simulink model "rfsoc4x2_ospfb_128"  (R2021a)
(part 3 of 339)

  pipeline45/1(q) -> q14/3(we)
  pipeline50/1(q) -> q15/1(addr)
  pipeline9/1(q) -> simple_bram_vacc3/1(new_acc)
  pipeline37/1(q) -> simple_bram_vacc1/2(din)
  Reinterpret5/1 -> pipeline11/1(d)
  Delay55/1 -> Delay92/1
  Reinterpret4/1 -> pipeline7/1(d)
  pipeline40/1(q) -> simple_bram_vacc5/1(new_acc)
  pipeline23/1(q) -> pipeline15/1(d)
  power8/1 -> Delay40/1
  Delay41/1 -> pipeline12/1(d)
  fft2/4(out02) -> Delay38/1
  pipeline43/1(q) -> simple_bram_vacc6/2(din)
  simple_bram_vacc6/2(valid) -> pipeline45/1(d)
  pipeline7/1(q) -> q16/2(data_in)
  Delay97/1 -> pipeline70/1(d)
  Delay91/1 -> pipeline39/1(d)
  q9/1(data_out) -> Terminator17/1
  Delay46/1 -> power8/1
  simple_bram_vacc4/2(valid) -> pipeline52/1(d)
  Delay93/1 -> pipeline8/1(d)
  [new_acc] -> pipeline9/1(d)
  simple_bram_vacc7/1(dout) -> Reinterpret2/1
  fft2/3(out01) -> Delay36/1
  fft2/7(out05) -> Delay53/1
  simple_bram_vacc6/1(dout) -> Reinterpret6/1
  pipeline51/1(q) -> q15/2(data_in)
  pipeline47/1(q) -> pipeline41/1(d)
  [new_acc] -> pipeline32/1(d)
  q10/1(data_out) -> Terminator9/1
  Reinterpret8/1 -> pipeline51/1(d)
  pipeline33/1(q) -> simple_bram_vacc2/2(din)
  simple_bram_vacc4/1(dout) -> Reinterpret4/1
  Delay44/1 -> Delay39/1
  q11/1(data_out) -> Terminator10/1
  spect_cnt1/1 -> pipeline29/1(d), pipeline22/1(d), pipeline30/1(d), pipeline53/1(d), pipeline46/1(d), pipeline59/1(d), pipeline50/1(d), pipeline26/1(d)
  Reinterpret2/1 -> pipeline38/1(d)
  [new_acc] -> pipeline16/1(d)
  power6/1 -> Delay97/1
  [new_acc] -> pipeline40/1(d)
  Delay42/1 -> power2/1
  simple_bram_vacc1/2(valid) -> pipeline25/1(d)
  simple_bram_vacc3/1(dout) -> Reinterpret8/1
  Delay92/1 -> power5/1
  Delay32/1 -> Delay44/1
  pipeline6/1(q) -> simple_bram_vacc4/2(din)
  [new_acc] -> pipeline14/1(d)
  [acc_len] -> acc_cntrl1/1(acc_len)
  pipeline5/1(q) -> simple_bram_vacc4/1(new_acc)
  pipeline26/1(q) -> q11/1(addr)
  Delay38/1 -> Delay42/1
  pipeline28/1(q) -> q12/3(we)
  Delay96/1 -> power6/1
  Delay53/1 -> Delay54/1
  fft2/9(out07) -> Delay95/1
  pipeline16/1(q) -> simple_bram_vacc16/1(new_acc)
  Delay48/1 -> power3/1
  pipeline31/1(q) -> pipeline33/1(d)
  Delay40/1 -> pipeline23/1(d)
  Delay52/1 -> Delay94/1
  pipeline25/1(q) -> q11/3(we)
  pipeline32/1(q) -> simple_bram_vacc2/1(new_acc)
  power1/1 -> Delay41/1
  simple_bram_vacc2/1(dout) -> Reinterpret1/1
  Delay35/1 -> Delay46/1
  pipeline8/1(q) -> pipeline10/1(d)
  Delay51/1 -> pipeline31/1(d)
  pipeline15/1(q) -> simple_bram_vacc7/2(din)
  pipeline48/1(q) -> q14/2(data_in)
  power4/1 -> Delay91/1
  power7/1 -> Delay56/1
  simple_bram_vacc5/2(valid) -> pipeline44/1(d)
  simple_bram_vacc5/1(dout) -> Reinterpret5/1
  q13/1(data_out) -> Terminator44/1
  simple_bram_vacc16/1(dout) -> Reinterpret3/1
  power2/1 -> Delay45/1
  fft2/8(out06) -> Delay55/1
  pipeline53/1(q) -> q13/1(addr)
  pipeline42/1(q) -> simple_bram_vacc6/1(new_acc)
  pipeline41/1(q) -> simple_bram_vacc5/2(din)
  q15/1(data_out) -> Terminator36/1
  Delay47/1 -> Delay48/1
  pipeline21/1(q) -> q10/3(we)
  power5/1 -> Delay93/1
  pipeline29/1(q) -> q9/1(addr)
  pipeline39/1(q) -> pipeline43/1(d)
  q14/1(data_out) -> Terminator35/1
  pipeline44/1(q) -> q13/3(we)
  power3/1 -> Delay51/1
  acc_cntrl1/1(new_acc) -> [new_acc]
  Delay95/1 -> Delay96/1
  q12/1(data_out) -> Terminator13/1
  fft2/2(out00) -> Delay35/1
  pipeline36/1(q) -> simple_bram_vacc1/1(new_acc)
  pipeline27/1(q) -> q11/2(data_in)
  Delay37/1 -> power1/1
  munge3/1(dout) -> bus_expand6/1(bus_in)
  bus_expand6/3(out6) -> fft2/5(in02)
  bus_expand6/4(out5) -> fft2/6(in03)
  bus_expand6/6(out3) -> fft2/8(in05)
  bus_expand6/1(msb_out8) -> fft2/3(in00)
  bus_expand6/8(lsb_out1) -> fft2/10(in07)
  [pfb1_sync] -> Delay43/1
  Delay43/1 -> fft2/1(sync)
  Constant60/1 -> fft2/2(shift)
  bus_expand6/7(out2) -> fft2/9(in06)
  fft2/10(of) -> Terminator45/1
  bus_expand6/2(out7) -> fft2/4(in01)
  bus_expand6/5(out4) -> fft2/7(in04)
  Delay31/1 -> Mux4/1
  [ram3_out1] -> Mux4/2
  Mux4/1 -> munge3/1(din)
  [ram3_out8] -> Mux4/9
  [ram3_out2] -> Mux4/3
  [ram3_out4] -> Mux4/5
  [ram3_out7] -> Mux4/8
  [ram3_out5] -> Mux4/6
  [mux_sel] -> Delay31/1
  [ram3_out3] -> Mux4/4
  [ram3_out6] -> Mux4/7
  Constant54/1 -> Dual Port RAM15/6
  Dual Port RAM15/2 -> [ram3_out5]
  Dual Port RAM18/2 -> [ram3_out3]
  [read_addr3] -> Dual Port RAM10/4
  [pfb_out3] -> Dual Port RAM18/2
  [write_addr3] -> Dual Port RAM17/1
  Constant53/1 -> Dual Port RAM15/5
  Constant34/1 -> Dual Port RAM9/6
  Dual Port RAM8/1 -> Terminator15/1
  Dual Port RAM16/1 -> Terminator14/1
  [write_addr3] -> Dual Port RAM18/1
  Constant58/1 -> Dual Port RAM7/5
  Dual Port RAM9/2 -> [ram3_out8]
  [write_addr3] -> Dual Port RAM8/1
  [pfb_out2] -> Dual Port RAM17/2
  Dual Port RAM7/1 -> Terminator5/1
  [read_addr3] -> Dual Port RAM7/4
  Constant33/1 -> Dual Port RAM9/5
  [pfb_out1] -> Dual Port RAM7/2
  Constant52/1 -> Dual Port RAM15/3
  [read_addr3] -> Dual Port RAM9/4
  Constant31/1 -> Dual Port RAM8/6
  Constant57/1 -> Dual Port RAM7/3
  Constant61/1 -> Dual Port RAM17/3
  Constant27/1 -> Dual Port RAM10/6
  [write_addr3] -> Dual Port RAM10/1
  Dual Port RAM8/2 -> [ram3_out7]
  Constant7/1 -> Dual Port RAM8/3
  [pfb_out7] -> Dual Port RAM8/2
  [write_addr3] -> Dual Port RAM16/1
  Dual Port RAM7/2 -> [ram3_out1]
  Dual Port RAM10/1 -> Terminator42/1
  Constant26/1 -> Dual Port RAM10/5
  [pfb_out5] -> Dual Port RAM15/2
  [write_addr3] -> Dual Port RAM9/1
  Constant36/1 -> Dual Port RAM16/6
  Constant22/1 -> Dual Port RAM8/5
  Constant56/1 -> Dual Port RAM17/6
  [read_addr3] -> Dual Port RAM16/4
  Dual Port RAM10/2 -> [ram3_out4]
  Constant23/1 -> Dual Port RAM18/5
  [pfb_out8] -> Dual Port RAM9/2
  Dual Port RAM16/2 -> [ram3_out6]
  Constant32/1 -> Dual Port RAM9/3
  Constant62/1 -> Dual Port RAM16/3
  Dual Port RAM17/2 -> [ram3_out2]
  Dual Port RAM9/1 -> Terminator39/1
  [write_addr3] -> Dual Port RAM7/1
  [read_addr3] -> Dual Port RAM15/4
  Dual Port RAM18/1 -> Terminator41/1
  [read_addr3] -> Dual Port RAM18/4
  Constant59/1 -> Dual Port RAM7/6
  [read_addr3] -> Dual Port RAM17/4
  [write_addr3] -> Dual Port RAM15/1
  Constant5/1 -> Dual Port RAM18/3
  Constant35/1 -> Dual Port RAM16/5
  Constant25/1 -> Dual Port RAM10/3
  [read_addr3] -> Dual Port RAM8/4
  Constant55/1 -> Dual Port RAM17/5
  Dual Port RAM15/1 -> Terminator43/1
  Dual Port RAM17/1 -> Terminator40/1
  [pfb_out6] -> Dual Port RAM16/2
  Constant24/1 -> Dual Port RAM18/6
  [pfb_out4] -> Dual Port RAM10/2
  [pfb1_sync] -> Counter21/1, Counter30/1
  [pfb1_sync] -> Counter22/1
  edge_detect10/1(out) -> Logical1/2
  edge_detect8/1(out) -> Logical6/2
  Counter22/1 -> Delay30/1
  Counter30/1 -> [mux_sel]
  [pfb1_sync] -> Counter28/1, Counter27/1
  Logical5/1 -> Counter26/2
  Counter29/1 -> Slice7/1
  Slice10/1 -> edge_detect10/1(in)
  edge_detect9/1(out) -> Logical7/2
  AddSub4/1 -> [write_addr3]
  [pfb1_sync] -> Counter24/1, Counter23/1
  Counter20/1 -> Delay29/1
  [en_ctrl2] -> Logical7/1
  Counter24/1 -> Slice9/1
  Logical1/1 -> Counter30/2
  [pfb1_sync] -> Counter29/1, Counter26/1
  Counter27/1 -> AddSub4/1
  Slice7/1 -> edge_detect7/1(in)
  [en_ctrl2] -> Logical6/1
  Logical6/1 -> Counter27/2
  [en_ctrl2] -> Logical1/1
  Slice8/1 -> edge_detect8/1(in)
  Counter21/1 -> Slice10/1
  Counter28/1 -> Slice8/1
  [en_ctrl2] -> Logical5/1
  Delay29/1 -> AddSub5/2
  Delay30/1 -> AddSub6/2
  Slice9/1 -> edge_detect9/1(in)
  edge_detect7/1(out) -> Logical5/2
  [pfb1_sync] -> Counter20/1
  Counter26/1 -> AddSub5/1
  AddSub5/1 -> AddSub4/2
  Logical7/1 -> Counter23/2
  AddSub6/1 -> [read_addr3]
  Counter23/1 -> AddSub6/1
  fft_wideband_real1/9(out07) -> Delay28/1
  fft_wideband_real1/8(out06) -> Delay27/1
  Delay24/1 -> [pfb_out5]
  bus_expand5/14(out3) -> fft_wideband_real1/16(in013)
  bus_expand5/10(out7) -> fft_wideband_real1/12(in09)
  bus_expand5/2(out15) -> fft_wideband_real1/4(in01)
  bus_expand5/16(lsb_out1) -> fft_wideband_real1/18(in015)
  Delay19/1 -> [pfb_out2]
  bus_expand5/5(out12) -> fft_wideband_real1/7(in04)
  Delay26/1 -> [pfb_out6]
  [pff1_sync] -> Delay18/1
  Delay27/1 -> [pfb_out7]
  Delay28/1 -> [pfb_out8]
  bus_expand5/11(out6) -> fft_wideband_real1/13(in010)
  Delay20/1 -> [pfb_out3]
  fft_wideband_real1/2(out00) -> Delay7/1
  Delay22/1 -> [pfb_out4]
  bus_expand5/15(out2) -> fft_wideband_real1/17(in014)
  fft_wideband_real1/6(out04) -> Delay24/1
  bus_expand5/4(out13) -> fft_wideband_real1/6(in03)
  fft_wideband_real1/5(out03) -> Delay22/1
  bus_expand5/1(msb_out16) -> fft_wideband_real1/3(in00)
  bus_expand5/6(out11) -> fft_wideband_real1/8(in05)
  bus_expand5/3(out14) -> fft_wideband_real1/5(in02)
  fft_wideband_real1/4(out02) -> Delay20/1
  bus_expand5/12(out5) -> fft_wideband_real1/14(in011)
  Delay18/1 -> fft_wideband_real1/1(sync)
  bus_expand5/7(out10) -> fft_wideband_real1/9(in06)
  [ram2_out] -> bus_expand5/1(bus_in)
  Constant4/1 -> fft_wideband_real1/2(shift)
  fft_wideband_real1/10(of) -> Terminator46/1
  bus_expand5/8(out9) -> fft_wideband_real1/10(in07)
  bus_expand5/9(out8) -> fft_wideband_real1/11(in08)
  fft_wideband_real1/3(out01) -> Delay19/1
  Delay7/1 -> [pfb_out1]
  fft_wideband_real1/1(sync_out) -> [pfb1_sync]
  bus_expand5/13(out4) -> fft_wideband_real1/15(in012)
  fft_wideband_real1/7(out05) -> Delay26/1
  bus_create5/1(bus_out) -> [current_data]
  bus_expand1/1(msb_out12) -> bus_create5/1(in1)
  bus_expand1/2(out11) -> bus_create5/2(in2)
  bus_expand1/3(out10) -> bus_create5/3(in3)
  bus_expand1/4(out9) -> bus_create5/4(in4)
  bus_expand1/5(out8) -> bus_create5/5(in5)
  bus_expand1/6(out7) -> bus_create5/6(in6)
  bus_expand1/7(out6) -> bus_create5/7(in7)
  bus_expand1/8(out5) -> bus_create5/8(in8)
  bus_expand1/9(out4) -> bus_create5/9(in9)
  bus_expand1/10(out3) -> bus_create5/10(in10)
  bus_expand1/11(out2) -> bus_create5/11(in11)
  bus_expand1/12(lsb_out1) -> bus_create5/12(in12)
  Delay102/1 -> AddSub7/1
  munge5/1(dout) -> mux_2/1(bus_in)
  [sync_gen] -> Counter33/1
  Slice13/1 -> Concat3/1
  Delay103/1 -> Relational3/1
  Constant67/1 -> Dual Port RAM19/7
  Dual Port RAM19/1 -> [ram_outa]
  Concat3/1 -> [c2]
  Concat9/1 -> [c3]
  [write_en] -> Logical8/2
  [current_data] -> Delay98/1
  Slice12/1 -> Delay100/1
  Delay98/1 -> Concat2/2
  Counter36/1 -> Slice18/1
  [c1] -> Mux6/3
  [sync_gen] -> Counter34/1
  Counter31/1 -> Delay103/1
  Mux6/1 -> [os_data]
  Constant64/1 -> Relational1/2
  [sync_gen] -> Counter31/1
  Dual Port RAM19/2 -> [ram_outb]
  Constant69/1 -> AddSub8/2
  Convert4/1 -> [en_ctrl]
  [current_data] -> Concat9/1
  Counter35/1 -> AddSub7/2
  Relational2/1 -> Mux7/1
  Constant66/1 -> Dual Port RAM19/6
  [sync_gen] -> Counter32/1
  Counter32/1 -> Delay101/1
  Logical8/1 -> Counter33/2
  Slice11/1 -> Concat2/1
  [os_data] -> Dual Port RAM19/2
  AddSub7/1 -> AddSub8/1, Mux7/2, Relational2/1
  [en_ctrl] -> Logical8/1
  Concat2/1 -> [c1]
  Logical11/1 -> Counter35/2
  Slice14/1 -> Delay99/1
  [write_addr] -> Dual Port RAM19/1
  [current_data] -> Slice14/1, Slice13/1
  Constant68/1 -> Relational2/2
  [read_addr] -> Dual Port RAM19/4
  Relational3/1 -> [ram_out_sel]
  Counter33/1 -> [write_addr]
  Constant65/1 -> Dual Port RAM19/5
  Delay99/1 -> Concat9/2
  [write_en] -> Dual Port RAM19/3
  edge_detect11/1(out) -> Logical11/2
  Delay100/1 -> Concat3/2
  Mux7/1 -> [read_addr]
  Constant63/1 -> Mux6/2
  [c3] -> Mux6/5
  [sync_gen] -> Counter37/1
  [sync_gen] -> Counter35/1, Counter36/1
  [c2] -> Mux6/4
  [current_data] -> Slice12/1, Slice11/1
  Delay101/1 -> Relational1/1, Mux6/1
  Relational1/1 -> [write_en]
  Counter34/1 -> Convert4/1
  Constant70/1 -> Relational3/2
  Counter37/1 -> Delay102/1
  [en_ctrl] -> Logical11/1
  Slice18/1 -> edge_detect11/1(in)
  AddSub8/1 -> Mux7/3
  [sync_gen] -> pipeline77/1(d)
  mux_2/5(out12) -> pfb_fir_real11/6(pol1_in5)
  mux_2/12(out5) -> pfb_fir_real11/13(pol1_in12)
  mux_2/13(out4) -> pfb_fir_real11/14(pol1_in13)
  mux_2/9(out8) -> pfb_fir_real11/10(pol1_in9)
  pipeline77/1(q) -> pfb_fir_real11/1(sync)
  mux_2/15(out2) -> pfb_fir_real11/16(pol1_in15)
  mux_2/7(out10) -> pfb_fir_real11/8(pol1_in7)
  mux_2/1(msb_out16) -> pfb_fir_real11/2(pol1_in1)
  [en_ctrl] -> pfb_fir_real11/18(en_ctrl)
  mux_2/16(lsb_out1) -> pfb_fir_real11/17(pol1_in16)
  mux_2/2(out15) -> pfb_fir_real11/3(pol1_in2)
  mux_2/4(out13) -> pfb_fir_real11/5(pol1_in4)
  mux_2/11(out6) -> pfb_fir_real11/12(pol1_in11)
  mux_2/10(out7) -> pfb_fir_real11/11(pol1_in10)
  mux_2/14(out3) -> pfb_fir_real11/15(pol1_in14)
  mux_2/3(out14) -> pfb_fir_real11/4(pol1_in3)
  mux_2/6(out11) -> pfb_fir_real11/7(pol1_in6)
  mux_2/8(out9) -> pfb_fir_real11/9(pol1_in8)
  pfb_fir_real11/1(sync_out) -> [pff1_sync]
  [pff1_sync] -> Counter39/1, Counter38/1
  Delay105/1 -> [write_addr2]
  [pff1_sync] -> Counter42/1
  [pff1_sync] -> Counter40/1
  Counter41/1 -> Delay105/1
  [pff1_sync] -> Counter44/1, Counter43/1
  Counter44/1 -> Slice21/1
  Dual Port RAM20/1 -> Terminator47/1
  Counter43/1 -> AddSub9/1
  AddSub14/1 -> Relational13/1, Mux14/2, AddSub15/1
  [write_addr2] -> Dual Port RAM20/1
  Logical13/1 -> Counter43/2
  Slice21/1 -> edge_detect13/1(in)
  Constant72/1 -> Dual Port RAM20/5
  Mux14/1 -> AddSub9/2
  Counter39/1 -> Slice19/1
  Dual Port RAM20/2 -> [ram2_out]
  Delay104/1 -> AddSub14/1
  Convert6/1 -> [en_ctrl1]
  Counter42/1 -> Convert6/1
  Constant74/1 -> Relational13/2
  edge_detect12/1(out) -> Logical12/2
  edge_detect13/1(out) -> Logical13/2
  Counter40/1 -> Delay104/1
  Slice19/1 -> edge_detect12/1(in)
  [read_addr2] -> Dual Port RAM20/4
  [en_ctrl1] -> Logical12/1
  [en_ctrl1] -> Logical13/1
  AddSub9/1 -> [read_addr2]
  Relational13/1 -> Mux14/1
  Logical12/1 -> Counter38/2
  Counter38/1 -> AddSub14/2
  [dina] -> Dual Port RAM20/2
  AddSub15/1 -> Mux14/3
  Constant73/1 -> Dual Port RAM20/6
  Constant71/1 -> Dual Port RAM20/3
  [pff1_sync] -> Counter41/1
  Constant75/1 -> AddSub15/2
  pfb_fir_real11/8(pol1_out7) -> bus_create4/7(in7)
  pfb_fir_real11/12(pol1_out11) -> bus_create4/11(in11)
  Delay108/1 -> [dina]
  pfb_fir_real11/13(pol1_out12) -> bus_create4/12(in12)
  pfb_fir_real11/11(pol1_out10) -> bus_create4/10(in10)
  pfb_fir_real11/7(pol1_out6) -> bus_create4/6(in6)
  pfb_fir_real11/15(pol1_out14) -> bus_create4/14(in14)
  pfb_fir_real11/4(pol1_out3) -> bus_create4/3(in3)
  pfb_fir_real11/3(pol1_out2) -> bus_create4/2(in2)
  bus_create4/1(bus_out) -> Delay108/1
  pfb_fir_real11/6(pol1_out5) -> bus_create4/5(in5)
  pfb_fir_real11/14(pol1_out13) -> bus_create4/13(in13)
  pfb_fir_real11/16(pol1_out15) -> bus_create4/15(in15)
  pfb_fir_real11/5(pol1_out4) -> bus_create4/4(in4)
  pfb_fir_real11/10(pol1_out9) -> bus_create4/9(in9)
  pfb_fir_real11/9(pol1_out8) -> bus_create4/8(in8)
  pfb_fir_real11/2(pol1_out1) -> bus_create4/1(in1)
  pfb_fir_real11/17(pol1_out16) -> bus_create4/16(in16)
  [ram_outb] -> Mux12/3
  [ram_out_sel] -> Mux12/1
  [ram_outa] -> Mux12/2
  Mux12/1 -> [pff_in]
  [pff_in] -> munge5/1(din)
